simulink model "EINT_system_simulation"  (R2024a)
settings: Solver=FixedStepAuto  StartTime=0.0  StopTime=5  FixedStep=Ts  RelTol=1e-3
values from neighbouring files (symbols this model uses):
  Ts = 0.00001    (= 1e-05)    [random_init.m]
settings Model: Creator=Max  LastModifiedBy=rayan768
settings SolverCC: AlgebraicLoopSolver=TrustRegion
settings DebuggingCC: UnconnectedInputMsg=warning  UnconnectedOutputMsg=warning  UnconnectedLineMsg=warning
settings ModelReferenceCC: EnableRefExpFcnMdlSchedulingChecks=on
settings RTWCC: GPUComputeCapability=3.5
settings ConfigComp: CovMetricSettings=de  CovBoundaryAbsTol=1.0e-5

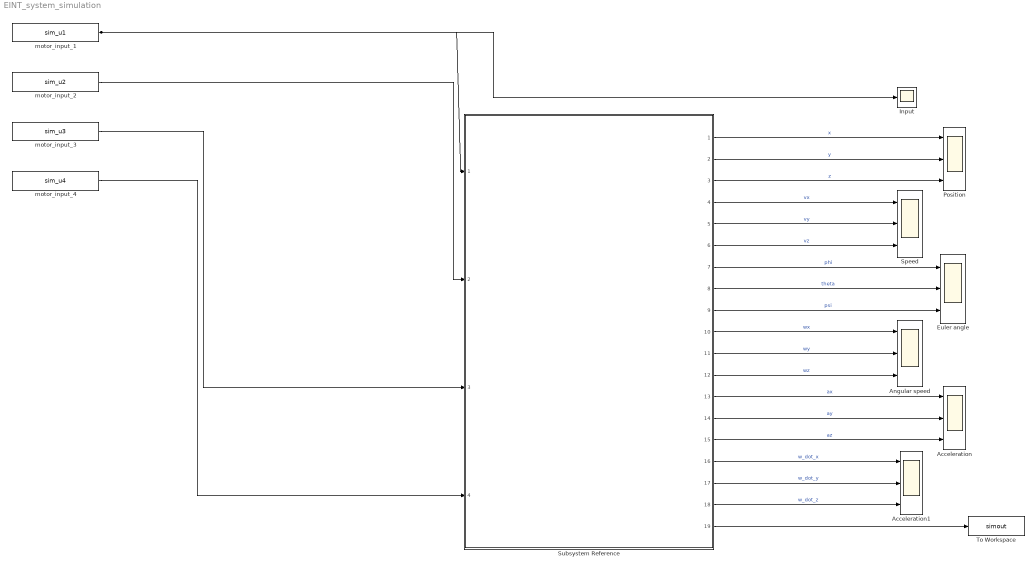
== system EINT_system_simulation ==
  Acceleration : Scope  NumInputPorts=3
  Acceleration1 : Scope  NumInputPorts=3
  Angular speed : Scope  NumInputPorts=3
  Euler angle : Scope  NumInputPorts=3
  Input : Scope
  Position : Scope  NumInputPorts=3
  Speed : Scope  NumInputPorts=3
  Subsystem Reference : Subsystem  ReferencedSubsystem=UAV_model
  To Workspace : ToWorkspace  VariableName=simout  SaveFormat=Structure With Time  SampleTime=Ts
  motor_input_1 : FromWorkspace  VariableName=sim_u1  SampleTime=Ts  Interpolate=off  OutputAfterFinalValue=Holding final value
  motor_input_2 : FromWorkspace  VariableName=sim_u2  SampleTime=Ts  Interpolate=off  OutputAfterFinalValue=Holding final value
  motor_input_3 : FromWorkspace  VariableName=sim_u3  SampleTime=Ts  Interpolate=off  OutputAfterFinalValue=Holding final value
  motor_input_4 : FromWorkspace  VariableName=sim_u4  SampleTime=Ts  Interpolate=off  OutputAfterFinalValue=Holding final value
  wires:
  Subsystem Reference/18 -> Acceleration1/3  "w_dot_z"
  Subsystem Reference/12 -> Angular speed/3  "wz"
  Subsystem Reference/17 -> Acceleration1/2  "w_dot_y"
  Subsystem Reference/9 -> Euler angle/3  "psi"
  Subsystem Reference/8 -> Euler angle/2  "theta"
  Subsystem Reference/14 -> Acceleration/2  "ay"
  Subsystem Reference/10 -> Angular speed/1  "wx"
  Subsystem Reference/2 -> Position/2  "y"
  Subsystem Reference/13 -> Acceleration/1  "ax"
  Subsystem Reference/15 -> Acceleration/3  "az"
  Subsystem Reference/16 -> Acceleration1/1  "w_dot_x"
  Subsystem Reference/7 -> Euler angle/1  "phi"
  Subsystem Reference/19 -> To Workspace/1
  Subsystem Reference/1 -> Position/1  "x"
  Subsystem Reference/6 -> Speed/3  "vz"
  Subsystem Reference/4 -> Speed/1  "vx"
  Subsystem Reference/3 -> Position/3  "z"
  Subsystem Reference/5 -> Speed/2  "vy"
  Subsystem Reference/11 -> Angular speed/2  "wy"
  motor_input_1/1 -> Subsystem Reference/1, Input/1
  motor_input_2/1 -> Subsystem Reference/2
  motor_input_3/1 -> Subsystem Reference/3
  motor_input_4/1 -> Subsystem Reference/4
